simulink model "model_1"  (R2023b)
settings: Solver=VariableStepAuto  StartTime=0.0  StopTime=10.0  RelTol=1e-3
model workspace (MATLAB code in the model file):
  | PRMTRS.VehicleMass = 5.0;
  | PRMTRS.VehicleInertiaTensor = diag([0.1 0.2 0.3]);
  | PRMTRS.PlanerSurface = 1.0;
  | 
  | 
  | PRMTRS.AirDensity = 0.8;
undefined symbols (not defined in the file or in its folder): A, Mot, Prop
libraries: matrix_library x2
settings Model: Creator=gogol  LastModifiedBy=gogol

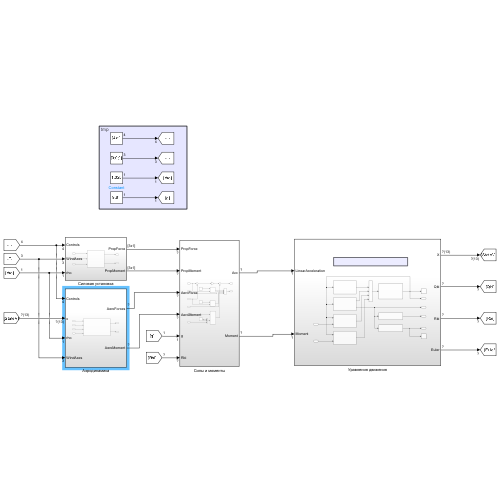
[thumbnail: Simulink's stored preview of the top-level diagram]
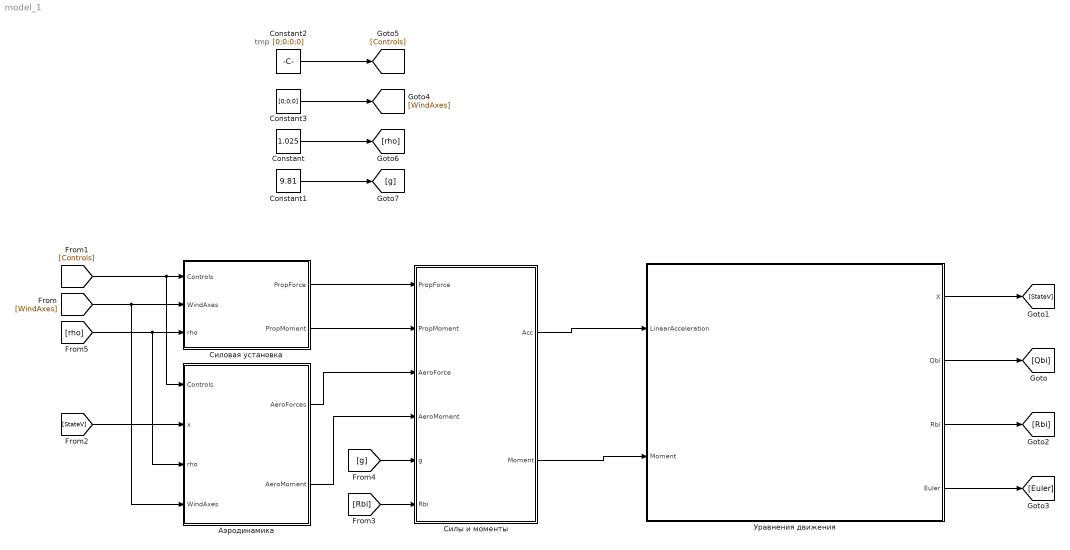
== system model_1 ==
  note: tmp
  Constant : Constant  Value=1.025
  Constant1 : Constant  Value=9.81
  Constant2 : Constant  Value=[0;0;0;0]
  Constant3 : Constant  Value=[0;0;0]
  Аэродинамика : Subsystem
  Силовая установка : Subsystem
  Силы и моменты : Subsystem
  Уравнения движения : Subsystem
  wires:
  Силы и моменты/1(Acc) -> Уравнения движения/1(LinearAcceleration)
  Силы и моменты/2(Moment) -> Уравнения движения/2(Moment)
  Аэродинамика/1(AeroForces) -> Силы и моменты/3(AeroForce)
  Аэродинамика/2(AeroMoment) -> Силы и моменты/4(AeroMoment)
  Силовая установка/1(PropForce) -> Силы и моменты/1(PropForce)
  Силовая установка/2(PropMoment) -> Силы и моменты/2(PropMoment)
  Уравнения движения/1(X) -> [StateV]
  Уравнения движения/2(Qbi) -> [Qbi]
  Уравнения движения/3(Rbi) -> [Rbi]
  Уравнения движения/4(Euler) -> [Euler]
  [WindAxes] -> Аэродинамика/4(WindAxes), Силовая установка/2(WindAxes)
  [Controls] -> Аэродинамика/1(Controls), Силовая установка/1(Controls)
  [StateV] -> Аэродинамика/2(x)
  [Rbi] -> Силы и моменты/6(Rbi)
  Constant2/1 -> [Controls]
  Constant3/1 -> [WindAxes]
  Constant/1 -> [rho]
  Constant1/1 -> [g]
  [g] -> Силы и моменты/5(g)
  [rho] -> Аэродинамика/3(rho), Силовая установка/3(rho)

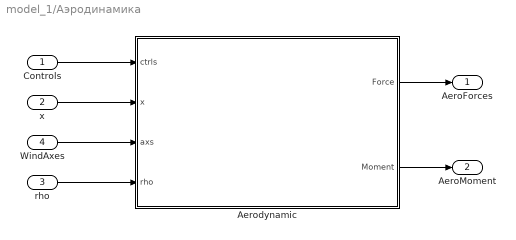
== system model_1/Аэродинамика ==
  Controls : Inport
  x : Inport  Port=2
  rho : Inport  Port=3
  WindAxes : Inport  Port=4
  Aerodynamic : MATLAB Function  TreatAsAtomicUnit=on
  AeroForces : Outport
  AeroMoment : Outport  Port=2
  wires:
  Controls/1 -> Aerodynamic/1(ctrls)
  WindAxes/1 -> Aerodynamic/3(axs)
  x/1 -> Aerodynamic/2(x)
  rho/1 -> Aerodynamic/4(rho)
  Aerodynamic/1(Force) -> AeroForces/1
  Aerodynamic/2(Moment) -> AeroMoment/1

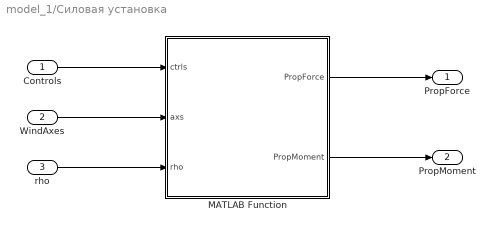
== system model_1/Силовая установка ==
  Controls : Inport
  WindAxes : Inport  Port=2
  rho : Inport  Port=3
  MATLAB Function : MATLAB Function  TreatAsAtomicUnit=on
  PropForce : Outport
  PropMoment : Outport  Port=2
  wires:
  Controls/1 -> MATLAB Function/1(ctrls)
  WindAxes/1 -> MATLAB Function/2(axs)
  rho/1 -> MATLAB Function/3(rho)
  MATLAB Function/1(PropForce) -> PropForce/1
  MATLAB Function/2(PropMoment) -> PropMoment/1

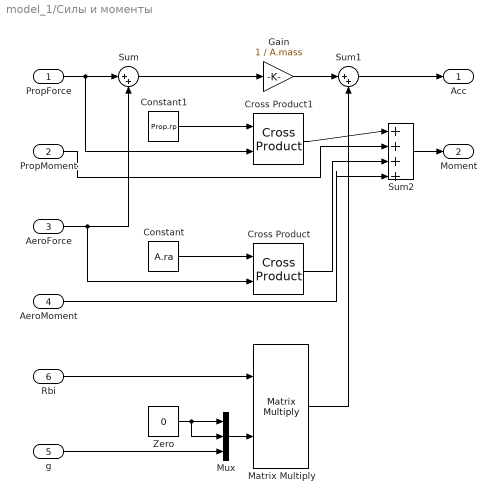
== system model_1/Силы и моменты ==
  PropForce : Inport
  PropMoment : Inport  Port=2
  AeroForce : Inport  Port=3
  AeroMoment : Inport  Port=4
  g : Inport  Port=5
  Rbi : Inport  Port=6
  Constant : Constant  Value=A.ra
  Constant1 : Constant  Value=Prop.rp
  Cross Product : matrix_library/Cross Product
  Cross Product1 : matrix_library/Cross Product
  Gain : Gain  Gain=1 / A.mass
  Matrix Multiply : Product  Multiplication=Matrix(*)
  Mux : Mux  Inputs=3
  Sum : Sum  Inputs=|++
  Sum1 : Sum  Inputs=|++
  Sum2 : Sum  Inputs=|++++
  Zero : Constant  Value=0  OutDataTypeStr=Inherit: Inherit via back propagation
  Acc : Outport
  Moment : Outport  Port=2
  wires:
  g/1 -> Mux/3
  Sum/1 -> Gain/1
  Sum1/1 -> Acc/1
  PropForce/1 -> Cross Product1/2, Sum/1
  AeroForce/1 -> Sum/2, Cross Product/2
  Gain/1 -> Sum1/1
  Rbi/1 -> Matrix Multiply/1
  Matrix Multiply/1 -> Sum1/2
  Mux/1 -> Matrix Multiply/2
  Zero/1 -> Mux/1, Mux/2
  Constant/1 -> Cross Product/1
  Constant1/1 -> Cross Product1/1
  Cross Product1/1 -> Sum2/1
  PropMoment/1 -> Sum2/2
  Cross Product/1 -> Sum2/3
  AeroMoment/1 -> Sum2/4
  Sum2/1 -> Moment/1

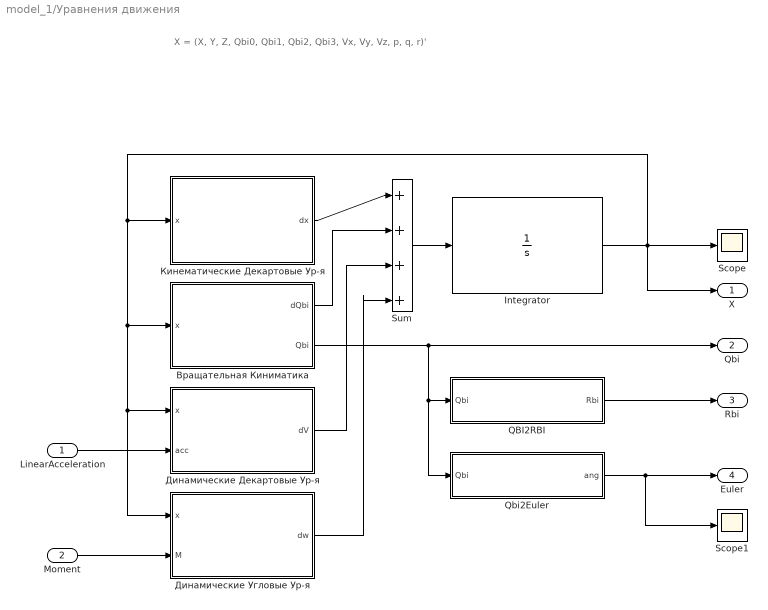
== system model_1/Уравнения движения ==
  note: X = (X, Y, Z, Qbi0, Qbi1, Qbi2, Qbi3, Vx, Vy, Vz, p, q, r)'
  LinearAcceleration : Inport
  Moment : Inport  Port=2
  Integrator : Integrator  InitialCondition=[0;0;0;0;1;0;0;1;0;0;0.05;0.05;0.05]
  QBI2RBI : MATLAB Function  TreatAsAtomicUnit=on
  Qbi2Euler : MATLAB Function  TreatAsAtomicUnit=on
  Scope : Scope
  Scope1 : Scope
  Sum : Sum  Inputs=|++++
  Вращательная Киниматика : MATLAB Function  TreatAsAtomicUnit=on
  Динамические Декартовые Ур-я : MATLAB Function  TreatAsAtomicUnit=on
  Динамические Угловые Ур-я : MATLAB Function  TreatAsAtomicUnit=on
  Кинематические Декартовые Ур-я : MATLAB Function  TreatAsAtomicUnit=on
  X : Outport
  Qbi : Outport  Port=2
  Rbi : Outport  Port=3
  Euler : Outport  Port=4
  wires:
  Integrator/1 -> X/1, Scope/1, Вращательная Киниматика/1(x), Динамические Угловые Ур-я/1(x), Динамические Декартовые Ур-я/1(x), Кинематические Декартовые Ур-я/1(x)
  Sum/1 -> Integrator/1
  Кинематические Декартовые Ур-я/1(dx) -> Sum/1
  Динамические Декартовые Ур-я/1(dV) -> Sum/3
  Динамические Угловые Ур-я/1(dw) -> Sum/4
  Вращательная Киниматика/1(dQbi) -> Sum/2
  Moment/1 -> Динамические Угловые Ур-я/2(M)
  LinearAcceleration/1 -> Динамические Декартовые Ур-я/2(acc)
  QBI2RBI/1(Rbi) -> Rbi/1
  Qbi2Euler/1(ang) -> Euler/1, Scope1/1
  Вращательная Киниматика/2(Qbi) -> Qbi2Euler/1(Qbi), QBI2RBI/1(Qbi), Qbi/1

== matlab function model_1/Уравнения движения/QBI2RBI ==
  data: Qbi input; Rbi output
function Rbi = Qbi2Rbi(Qbi)

q0 = Qbi(1);
q1 = Qbi(2);
q2 = Qbi(3);
q3 = Qbi(4);

Rbi = [q0^2 + q1^2 - q2^2 - q3^2, 2*(q1*q2 + q0*q3), 2*(q1*q3 - q0*q2)];
       [2*(q1*q2 - q0*q3), q0^2 - q1^2 + q2^2 - q3^2, 2*(q0*q1 + q2*q3)];
       [2*(q0*q2 + q1 * q3), 2*(q2 * q3 - q1* q0), q0^2 - q1^2 -q2^2 + q3^2];
end

== matlab function model_1/Уравнения движения/Кинематические Декартовые Ур-я ==
  data: x input; dx output
function dx = decard_kin(x)
    dx = zeros(13,1);
    dx(1:3) = x(7:9);
end

== matlab function model_1/Уравнения движения/Динамические Декартовые Ур-я ==
  data: x input; acc input; dV output
function dV = decard_dyn(x, acc)
    dV = zeros(13, 1);

   dV(8:10) = acc - cross(x(11:13), x(8:10));
end

== matlab function model_1/Уравнения движения/Динамические Угловые Ур-я ==
  data: x input; M input; dw output; PRMTRS parameter
function dw = angular_din(x, M, PRMTRS)
    dw = zeros(13,1);
    
    J = PRMTRS.VehicleInertiaTensor;
    w = x(11:13);
    dw(11:13) = inv(J) * (M - cross(w, J * w));
end

== matlab function model_1/Уравнения движения/Вращательная Киниматика ==
  data: x input; dQbi output; Qbi output
function [dQbi, Qbi]= QuaternionKinematics(x)
dQbi = zeros(13,1);

w = x(11:13);
Qbi = reshape(x(4:7), 4, 1);
norm = sqrt(Qbi(1)^2 + Qbi(2)^2 + Qbi(3)^2 + Qbi(4)^2);
Qbi = Qbi / norm;

A = [[0 -w(1) -w(2) -w(3)];
    [w(1) 0 w(3) -w(2)];
    [w(2) -w(3) 0 -w(1)];
    [w(3) w(2) -w(1) 0]];

dQbi(4:7) = 0.5 * (A*Qbi);
end

== matlab function model_1/Уравнения движения/Qbi2Euler ==
  data: Qbi input; ang output
function ang = Qbi2Euler(Qbi)
%ang = euler(Qbi', "ZYX", "frame");
ang = [0;0;0];
end

== matlab function model_1/Аэродинамика/Aerodynamic ==
  data: ctrls input; Force output; Moment output; x input; axs input; rho input; A parameter
function [Force, Moment] = AeroFMs(ctrls, x, axs, rho, A)

% ctrls = (da, de, dr, Vin)'
p = x(11); q = x(12); r = x(13);
Va = axs(1); % воздушная скорость
a = axs(2); % угол атаки
b = axs(3); % угол скольжения


% Аэродинамические коэффициенты
CL = A.CL0 + A.CLa * a + A.CLde*ctrls(2) + A.CLq*q*A.c / (2 * Va);
CD = A.CD0 + A.CDa * a + A.CDde*abs(ctrls(2)) + A.CDq*q*A.c / (2 * Va);
CY = A.CY0 + A.CYb * b + A.CYda * ctrls(1) + A.CYdr * ctrls(3) + ...
     + A.CYp * p * A.b / (2 * Va) + A.CYr * r * A.b / (2 * Va);

Cl = A.Cl0 + A.Clb * b + A.Clda * ctrls(1) + A.Cldr * ctrls(3) + A.Clp * p * A.b / (2 * Va) + ...
     + A.Clr * r * A.b / (2 * Va);
Cm = A.Cm0 + A.Cma * a + A.Cmde * ctrls(2) + A.Cmq * q * A.c / (2 * Va);
Cn = A.Cn0 + A.Cnb * b + A.Cnda * ctrls(1) + A.Cndr * ctrls(3) + A.Cnp * p * A.b / (2 * Va) + ...
     + A.Cnr * r * A.b / (2 * Va);

% Аэродинамические силы
ForceW = [-CD; CY; -CL] * A.S * (rho * Va^2) / 2
MomentW = [Cl * A.b; Cm * A.c; Cn * A.b] * A.S * (rho * Va^2) / 2

% Переход в ССК
Rbw = WindAxes2Rbw(axs);

Force = Rbw * ForceW;
Moment = Rbw * MomentW;
end

== matlab function model_1/Силовая установка/MATLAB Function ==
  data: PropForce output; PropMoment output; ctrls input; axs input; rho input; Prop parameter; Mot parameter
function [PropForce, PropMoment] = PropFMs(ctrls, axs, rho, Prop, Mot)

Vin = ctrls(4);

if (Vin == 0)
    PropForce = [0;0;0];
    PropMoment = [0;0;0];
    return
end

% Ветровая ССК stuff
Va  = axs(1);
a = axs(2); b = axs(3);
Rbw = WindAxes2Rbw(axs);

Va_body = Va * Rbw(1,1);

% Тяга
D = Prop.diameter;
a = rho * D^5 / (4 * pi^2) * Prop.CQ0;
b = rho * D^4 / (2 * pi) * Prop.CQ1 * Va + Mot.Kq * Mot.Kv / Mot.R;
c = rho * D^3 * Va^2  * Prop.CQ2 + Mot.Kq * Mot.i0 - Mot.Kq*Vin / Mot.R;

Omega = (-b + sqrt(b^2 - 4 * a * c)) / (2 * a);
if Omega < 0
    Omega = 0;
    J = 0;
else
    J = 2 * pi * Va / (Omega * D);
end

Thrust = rho*D^4/(4*pi^2)*Omega^2*(Prop.CT0 + Prop.CT1*J + Prop.CT2*J^2);
Torque = rho*D^5/(4*pi^2)*Omega^2*(Prop.CQ0 + Prop.CQ1*J + Prop.CQ2*J^2);

% Вывод в ССК

PropForce = [Thrust; 0; 0];
PropMoment = [-Torque; 0; 0];

end
